simulink model "Observer_Test_Live"  (R2026b)
settings: Solver=VariableStepAuto  StopTime=inf
undefined symbols (not defined in the file): Aobs, Bobs, Cobs, Dobs, du_min, ISCS_Ad, ISCS_Bd, ISCS_Cd, ISCS_Dd, ISCS_Tu, ISCS_Ty, P_on, Ts
settings Model: Creator=leont  LastModifiedBy=leont

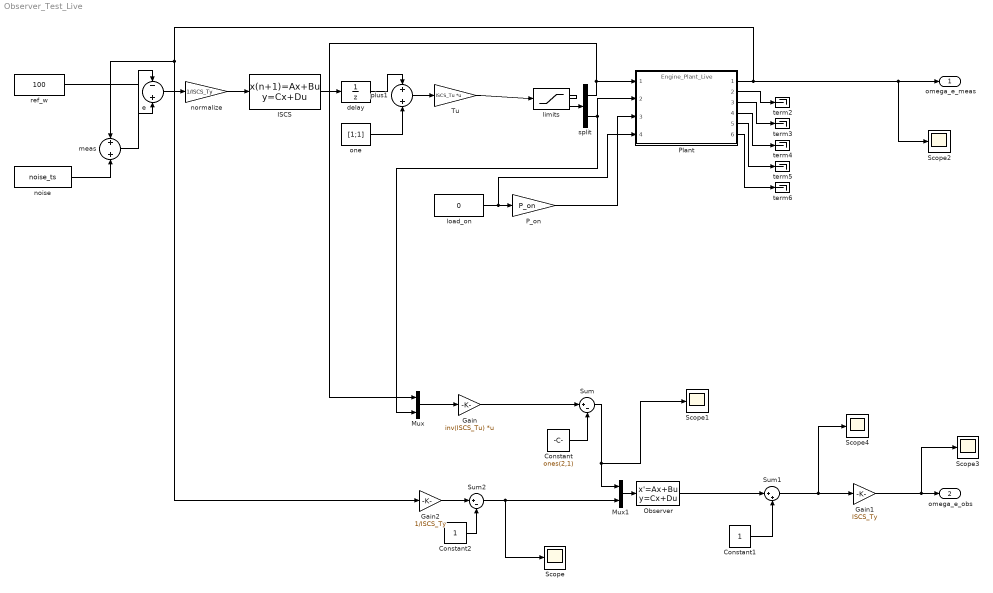
== system Observer_Test_Live ==
  Constant : Constant  Value=ones(2,1)
  Constant1 : Constant
  Constant2 : Constant
  Gain : Gain  Gain=inv(ISCS_Tu)  Multiplication=Matrix(K*u)
  Gain1 : Gain  Gain=ISCS_Ty
  Gain2 : Gain  Gain=1/ISCS_Ty
  ISCS : DiscreteStateSpace  A=ISCS_Ad  B=ISCS_Bd  C=ISCS_Cd  D=ISCS_Dd  InitialCondition=zeros(12,1)  SampleTime=Ts
  Mux : Mux  Inputs=2
  Mux1 : Mux  Inputs=2
  Observer : StateSpace  A=Aobs  B=Bobs  C=Cobs  D=Dobs  InitialCondition=0
  P_on : Gain  Gain=P_on
  Plant : ModelReference  ModelNameDialog=Engine_Plant_Live  SimulationMode=Normal  ModelReferenceVersion=1.25
  Scope{,1..4} (5 alike) : Scope
      Scope settings: ActiveDisplayYMinimum=-0.0025533610261974926  ActiveDisplayYMaximum=0.0027493841960254117
      Scope1 settings: ActiveDisplayYMinimum=-1.1696912140251245  ActiveDisplayYMaximum=1.5844647872137192
      Scope2 settings: ActiveDisplayYMinimum=-9.220186429408642  ActiveDisplayYMaximum=124.68238114514418  DataLoggingVariableName=ScopeData2
      Scope3 settings: ActiveDisplayYMinimum=79.184380846513108  ActiveDisplayYMaximum=118.95394705469803  DataLoggingVariableName=ScopeData3
      Scope4 settings: ActiveDisplayYMinimum=-9.83375081396752  ActiveDisplayYMaximum=9.2138682336515245  DataLoggingVariableName=ScopeData4
  Sum : Sum  Inputs=|+-
  Sum1 : Sum  Inputs=|++
  Sum2 : Sum  Inputs=|+-
  Tu : Gain  Gain=ISCS_Tu  Multiplication=Matrix(K*u)
  delay : UnitDelay  InitialCondition=zeros(2,1)  SampleTime=Ts
  e : Sum  Inputs=-+
  limits : Saturate  UpperLimit=[100; 0]  LowerLimit=[0; du_min]
  load_on : Constant  Value=0
  meas : Sum
  noise : FromWorkspace  VariableName=noise_ts  SampleTime=Ts  Interpolate=off  OutputAfterFinalValue=Cyclic repetition
  normalize : Gain  Gain=1/ISCS_Ty
  one : Constant  Value=[1;1]
  plus1 : Sum
  ref_w : Constant  Value=100
  split : Demux  Outputs=2
  term{2..6} (5 alike) : Terminator
  omega_e_meas : Outport
  omega_e_obs : Outport  Port=2
  wires:
  Mux/1 -> Gain/1
  Constant/1 -> Sum/2
  Gain/1 -> Sum/1
  Sum1/1 -> Scope4/1, Gain1/1
  Constant1/1 -> Sum1/2
  Observer/1 -> Sum1/1
  Gain2/1 -> Sum2/1
  Constant2/1 -> Sum2/2
  Gain1/1 -> Scope3/1, omega_e_obs/1
  Plant/4 -> term4/1
  one/1 -> plus1/2
  ref_w/1 -> e/2
  plus1/1 -> Tu/1
  meas/1 -> e/1
  Plant/5 -> term5/1
  delay/1 -> plus1/1
  P_on/1 -> Plant/3
  limits/1 -> split/1
  noise/1 -> meas/2
  e/1 -> normalize/1
  Plant/2 -> term2/1
  load_on/1 -> P_on/1, Plant/4
  Plant/6 -> term6/1
  split/1 -> Mux/1, Plant/1
  Plant/1 -> Gain2/1, meas/1, Scope2/1, omega_e_meas/1
  normalize/1 -> ISCS/1
  Plant/3 -> term3/1
  Tu/1 -> limits/1
  ISCS/1 -> delay/1
  split/2 -> Plant/2, Mux/2
  Sum/1 -> Scope1/1, Mux1/1
  Mux1/1 -> Observer/1
  Sum2/1 -> Scope/1, Mux1/2
